simulink model "CartIdentPiMod2"  (R2025b)
settings: Solver=ode1  StartTime=0.0  StopTime=20  FixedStep=0.001  RelTol=1e-3  EnableMultiTasking=on
undefined symbols (not defined in the file): MQTTsample
libraries: raspberrypiCommlib x2, raspberrypiBasiclib x1, simulink x1, raspberrypiIOTlib x1
settings Model: SimulationMode=external  ExtModeTrigMode=oneshot  ExtModeTrigDuration=100000  Creator=Demo11  LastModifiedBy=brfon_9d4n8nc
settings SolverCC: AlgebraicLoopSolver=TrustRegion  PositivePriorityOrder=on  AutoInsertRateTranBlk=on
settings DataIOCC: SaveFormat=Array  SignalLoggingSaveFormat=ModelDataLogs  ReturnWorkspaceOutputs=off  SignalLoggingName=sigsOut
settings OptimizationCC: BlockReduction=off  BooleanDataType=off  EnhancedBackFolding=on  PassReuseOutputArgsAs=Individual arguments  ExpressionDepthLimit=2147483647.0  ZeroExternalMemoryAtStartup=off  ZeroInternalMemoryAtStartup=off  InitFltsAndDblsToZero=on  MaxStackSize=200000  OptimizeBlockOrder=speed  DifferentSizesBufferReuse=on  OptimizationCustomize=off  EfficientTunableParamExpr=on
settings DebuggingCC: SaveWithParameterizedLinksMsg=none  UnderspecifiedInitializationDetection=Classic  MergeDetectMultiDrivingBlocksExec=none  SignalResolutionControl=TryResolveAllWithWarning  MultiTaskDSMMsg=warning  MultiTaskCondExecSysMsg=none  ParameterTunabilityLossMsg=error  FcnCallInpInsideContextMsg=warning  UnconnectedInputMsg=warning  UnconnectedOutputMsg=warning  UnconnectedLineMsg=warning  AllowSymbolicDim=off  StateNameClashWarn=warning  SFUnexpectedBacktrackingDiag=warning  SFNoUnconditionalDefaultTransitionDiag=warning  SFExecutionAtInitializationDiag=none  ArithmeticOperatorsInVariantConditions=warning
settings HardwareCC: ProdBitPerLong=64.0  ProdLargestAtomicInteger=LongLong  ProdLargestAtomicFloat=Double  ProdLongLongMode=on  ProdHWDeviceType=ARM Compatible->ARM Cortex-A (64-bit)  TargetBitPerLong=64.0  TargetBitPerPointer=64.0  TargetIntDivRoundTo=Zero  TargetEndianess=LittleEndian  TargetWordSize=64.0  TargetHWDeviceType=Intel->x86-64
settings ModelReferenceCC: EnableRefExpFcnMdlSchedulingChecks=on  PropagateSignalLabelsOutOfModel=off
settings SFSimCC: SimUseLocalCustomCode=off  CustomCodeUndefinedFunction=UseInterfaceOnly
settings RTWCC: SystemTargetFile=ert.tlc  HardwareBoard=Raspberry Pi (64bit)  TLCOptions="-aInlineSetEventsForThisBaseRateFcn=TLC_FALSE -aSuppressMultiTaskScheduler=TLC_FALSE  -aRateBasedStepFcn=0"  TemplateMakefile=ert_default_tmf  RTWUseLocalCustomCode=off  Toolchain=GNU GCC Embedded Linux  BuildConfiguration=Faster Runs  GPUComputeCapability=3.5  Description=Embedded Coder
settings CodeAppCC: ForceParamTrailComments=on  IgnoreCustomStorageClasses=off  MaxIdLength=95.0  OperatorAnnotations=on  SimulinkDataObjDesc=on  SFDataObjDesc=on  InsertBlockDesc=on
settings ERTTargetCC: ExtModeTransport=2.0  ExtModeStaticAlloc=on  ExtModeMexFile=ext_xcp  ExtModeIntrfLevel=Level2 - Open  InlinedParameterPlacement=Hierarchical  CodeReplacementLibrary=ARM Cortex-A CMSIS  SupportContinuousTime=on  SupportVariableSizeSignals=on
settings ConfigComp: CovMetricSettings=dw  CovSaveCumulativeToWorkspaceVar=on  CovSaveSingleToWorkspaceVar=on  CovExternalEMLEnable=off

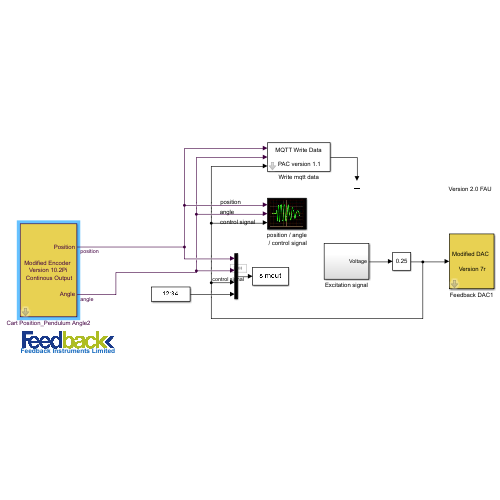
[thumbnail: Simulink's stored preview of the top-level diagram]
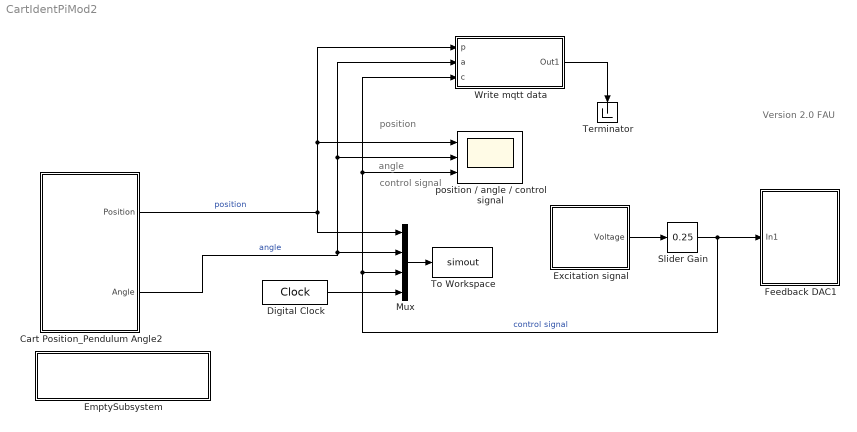
== system CartIdentPiMod2 ==
  note: position
  note: angle
  note: control signal
  note: Version 2.0 FAU
  Cart Position_Pendulum Angle2 : Subsystem  mask(Feedback Encoder Block){st=0.001, of1=0, of2=-1024}
      mask prompts: st "Sample Time"; of1 "Channel 1 Offset"; of2 "Channel 2 Offset"
      mask help: Special block to use with the Feedback experiments to read encoder channels using the digital I/O lines
      mask Display:
      | %image(imread('bckg.bmp'))
      | disp('Modified Encoder \nVersion 10.2Pi\n Continous Output')
      | port_label('output', 1, 'Position')
      | port_label('output', 2, 'Angle')
  Digital Clock : DigitalClock  SampleTime=0.001
  EmptySubsystem : Subsystem
      mask Display:
      | image(imread('FB-inst-blue2.jpg'))
      | disp('\n\nFeedback Instruments Limited')
  Excitation signal : Subsystem
  Feedback DAC1 : Subsystem  mask(DAC Unit for Feedback Experiments){st=0.001, ch=1}
      mask prompts: st "Sample Time"; ch "Output Channel"
      mask help:
      | Digital to Analog Output  for Feedback Experiments
      | using Advantech PCI1711  I/O board
      mask Display:
      | %image(imread('bckg.bmp'))
      | disp('Modified DAC \n\n Version 7r')
  Mux : Mux
  Slider Gain : simulink/Math Operations/Slider Gain  gain=0.25  low=-0.3  high=0.3
  Terminator : Terminator
  To Workspace : ToWorkspace  VariableName=simout  SampleTime=0.05
  Write mqtt data : Subsystem
      mask Display: disp('MQTT Write Data\n\n PAC version 1.1')
  position / angle / control signal : Scope  NumInputPorts=3
      settings: SampleTime=0.001  TimeSpan=20  ActiveDisplayYMinimum=-0.55  ActiveDisplayYMaximum=0.35  DataLoggingMaxPoints=100000  DataLoggingVariableName=ScopeData2
      mask Display: image(imread('scope.jpg'))
  wires:
  Cart Position_Pendulum Angle2/1(Position) -> Write mqtt data/1(p), position / angle / control signal/1, Mux/1  "position"
  Excitation signal/1(Voltage) -> Slider Gain/1
  Cart Position_Pendulum Angle2/2(Angle) -> Write mqtt data/2(a), position / angle / control signal/2, Mux/2  "angle"
  Slider Gain/1 -> Feedback DAC1/1(In1), Mux/3, Write mqtt data/3(c), position / angle / control signal/3  "control signal"
  Mux/1 -> To Workspace/1
  Digital Clock/1 -> Mux/4
  Write mqtt data/1(Out1) -> Terminator/1

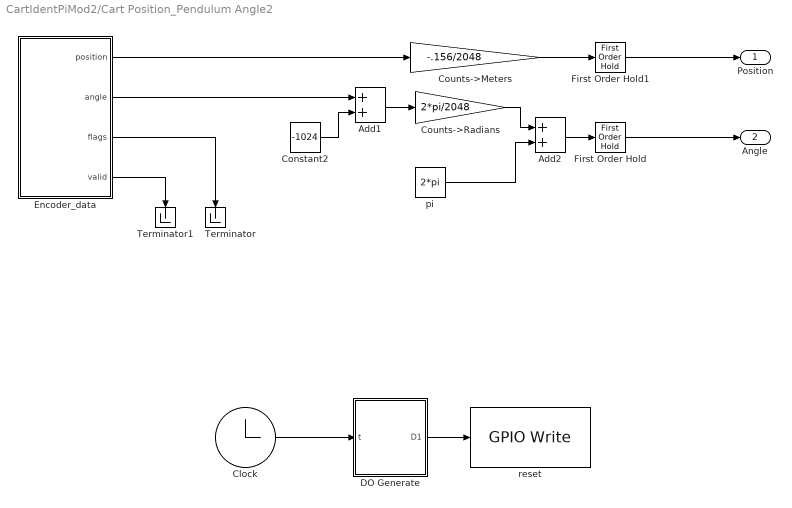
== system CartIdentPiMod2/Cart Position_Pendulum Angle2 ==
  Add1 : Sum
  Add2 : Sum
  Clock : Clock
  Constant2 : Constant  Value=-1024
  Counts->Meters : Gain  Gain=-.156/2048  SaturateOnIntegerOverflow=on  OutDataTypeStr=Inherit: Same as input  ParamDataTypeStr=Inherit: Same as input
  Counts->Radians : Gain  Gain=2*pi/2048  SaturateOnIntegerOverflow=on  OutDataTypeStr=Inherit: Same as input  ParamDataTypeStr=Inherit: Same as input
  DO Generate : MATLAB Function  TreatAsAtomicUnit=on
  Encoder_data : Subsystem
  First Order Hold : FirstOrderHold  OutputAlgorithm=Fast (Minimize Error)  ErrorTolerance=inf
  First Order Hold1 : FirstOrderHold  OutputAlgorithm=Fast (Minimize Error)  ErrorTolerance=inf
  Terminator : Terminator
  Terminator1 : Terminator
  pi : Constant  Value=2*pi
  reset : raspberrypiBasiclib/GPIO Write  BoardProperty=Pi 5 Model  gpio=6  blockPlatform=Raspberry Pi  PinNumber=17  board=[]  direction=[]
  Position : Outport
  Angle : Outport  Port=2
  wires:
  pi/1 -> Add2/2
  Counts->Radians/1 -> Add2/1
  Counts->Meters/1 -> First Order Hold1/1
  Clock/1 -> DO Generate/1(t)
  DO Generate/1(D1) -> reset/1
  Encoder_data/2(angle) -> Add1/1
  Encoder_data/1(position) -> Counts->Meters/1
  Add1/1 -> Counts->Radians/1
  Constant2/1 -> Add1/2
  Encoder_data/4(valid) -> Terminator1/1
  Encoder_data/3(flags) -> Terminator/1
  Add2/1 -> First Order Hold/1
  First Order Hold/1 -> Angle/1
  First Order Hold1/1 -> Position/1

== system CartIdentPiMod2/EmptySubsystem ==

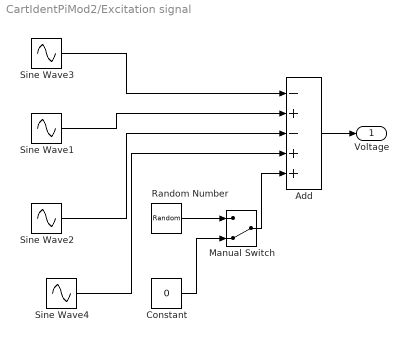
== system CartIdentPiMod2/Excitation signal ==
  Add : Sum  Inputs=-+-++
  Constant : Constant  Value=0
  Manual Switch : ManualSwitch  CurrentSetting=0
  Random Number : RandomNumber  Variance=0.1  SampleTime=0.1
  Sine Wave1 : Sin  Frequency=5  Phase=1  SampleTime=0
  Sine Wave2 : Sin  Frequency=15  SampleTime=0
  Sine Wave3 : Sin  Amplitude=0.5  Phase=0.5  SampleTime=0
  Sine Wave4 : Sin  Frequency=20  Phase=0.3  SampleTime=0
  Voltage : Outport
  wires:
  Add/1 -> Voltage/1
  Sine Wave3/1 -> Add/1
  Sine Wave1/1 -> Add/2
  Sine Wave2/1 -> Add/3
  Sine Wave4/1 -> Add/4
  Random Number/1 -> Manual Switch/1
  Manual Switch/1 -> Add/5
  Constant/1 -> Manual Switch/2

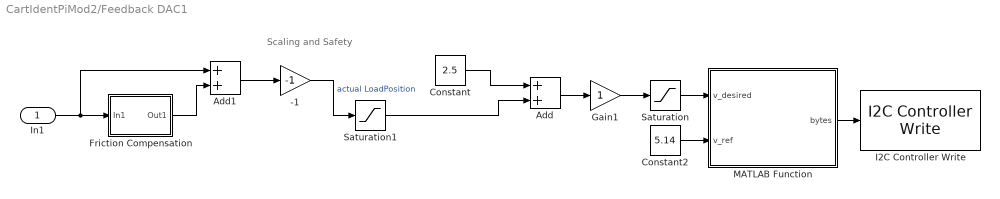
== system CartIdentPiMod2/Feedback DAC1 ==
  note: Scaling and Safety
  In1 : Inport
  -1 : Gain  Gain=-1  SaturateOnIntegerOverflow=on  OutDataTypeStr=Inherit: Same as input  ParamDataTypeStr=Inherit: Same as input
  Add : Sum  OutDataTypeStr=Inherit: Same as first input
  Add1 : Sum
  Constant : Constant  Value=2.5
  Constant2 : Constant  Value=5.14  SampleTime=-1
  Friction Compensation : Subsystem  mask(linear){frictionCompNeg=.1, frictionCompPos=.1}
      mask prompts: frictionCompNeg "Friction Compensation Magnitude in Negative Direction"; frictionCompPos "Friction Compensation Magnitude in Positive Direction"
      mask Display: plot(0,0,100,100,[40,30,20],[87,85,80],[46,54,54,46,46],[90,90,80,80,90],[46,45,45,46,54,55,55,54,46],[78,80,90,91,91,90,80,78,78],[51,51,49,49],[78,10,10,78],[90,80,70,60],[70,80,85,88],[20,10],[80,70],[20,20,15],[73,80,80],[85,80,80],[80,80,74])
  Gain1 : Gain
  I2C Controller Write : raspberrypiCommlib/I2C Controller Write  BoardProperty=Pi 5 Model  I2CModule=1  Mode=Master  SlaveAddress=0x60  SlaveByteOrder=BigEndian  Direction=Transmitter  RegisterAddressMode=off  RegisterAddress=0  SlaveDataType=uint8  DataLength=1  NoAck=off  RepeatedStart=off  OutputStatus=off
  MATLAB Function : MATLAB Function  TreatAsAtomicUnit=on
  Saturation : Saturate  UpperLimit=5.0  LowerLimit=0
  Saturation1 : Saturate  UpperLimit=2.5  LowerLimit=-2.5
  wires:
  MATLAB Function/1(bytes) -> I2C Controller Write/1
  Saturation/1 -> MATLAB Function/1(v_desired)
  Constant2/1 -> MATLAB Function/2(v_ref)
  Add1/1 -> -1/1
  -1/1 -> Saturation1/1  "actual LoadPosition"
  In1/1 -> Add1/1, Friction Compensation/1(In1)
  Friction Compensation/1(Out1) -> Add1/2
  Constant/1 -> Add/1
  Add/1 -> Gain1/1
  Gain1/1 -> Saturation/1
  Saturation1/1 -> Add/2

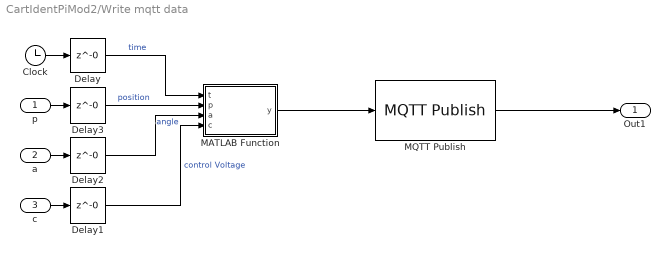
== system CartIdentPiMod2/Write mqtt data ==
  p : Inport
  a : Inport  Port=2
  c : Inport  Port=3
  Clock : Clock
  Delay{,1..3} (4 alike) : Delay  DelayLength=0  InitialCondition=0  SampleTime=MQTTsample
  MATLAB Function : MATLAB Function  TreatAsAtomicUnit=on
  MQTT Publish : raspberrypiIOTlib/MQTT Publish  Topic=raspi/to_django  QoS=0  RetainMsg=off  blockPlatform=RASPBERRYPI
  Out1 : Outport
  wires:
  MQTT Publish/1 -> Out1/1
  a/1 -> Delay2/1
  Clock/1 -> Delay/1
  Delay/1 -> MATLAB Function/1(t)  "time"
  p/1 -> Delay3/1
  Delay2/1 -> MATLAB Function/3(a)  "angle"
  c/1 -> Delay1/1
  Delay1/1 -> MATLAB Function/4(c)  "control Voltage"
  MATLAB Function/1(y) -> MQTT Publish/1
  Delay3/1 -> MATLAB Function/2(p)  "position"

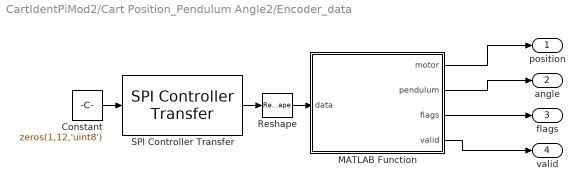
== system CartIdentPiMod2/Cart Position_Pendulum Angle2/Encoder_data ==
  Constant : Constant  Value=zeros(1,12,'uint8')
  MATLAB Function : MATLAB Function  TreatAsAtomicUnit=on
  Reshape : Reshape
  SPI Controller Transfer : raspberrypiCommlib/SPI Controller Transfer  BoardProperty=Pi 5 Model  SSPin=SPI0_CE0  SPIModule=uint32(0)  Mode=Master  BusSpeed=1000000  Pin=uint32(0)  FirstBitToTransfer=Most significant bit (MSB)  ClockMode=1  BlockFunction=Transfer  RegisterAddress=0  OutputDataType=int8  OutputDataLength=1
  position : Outport
  angle : Outport  Port=2
  flags : Outport  Port=3
  valid : Outport  Port=4
  wires:
  Constant/1 -> SPI Controller Transfer/1
  MATLAB Function/3(flags) -> flags/1
  SPI Controller Transfer/1 -> Reshape/1
  Reshape/1 -> MATLAB Function/1(data)
  MATLAB Function/2(pendulum) -> angle/1
  MATLAB Function/4(valid) -> valid/1
  MATLAB Function/1(motor) -> position/1

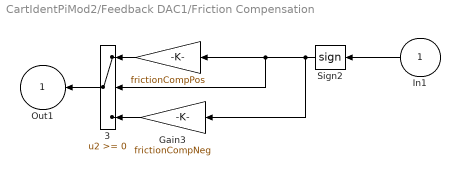
== system CartIdentPiMod2/Feedback DAC1/Friction Compensation ==
  In1 : Inport
  " " : Gain  Gain=frictionCompPos  SaturateOnIntegerOverflow=on  OutDataTypeStr=Inherit: Same as input  ParamDataTypeStr=Inherit: Same as input
  3 : Switch
  Gain3 : Gain  Gain=frictionCompNeg  SaturateOnIntegerOverflow=on  OutDataTypeStr=Inherit: Same as input  ParamDataTypeStr=Inherit: Same as input
  Sign2 : Signum  Tag=T
  Out1 : Outport  InitialOutput=0
  wires:
  3/1 -> Out1/1
  Sign2/1 -> 3/2, " "/1, Gain3/1
  Gain3/1 -> 3/3
  " "/1 -> 3/1
  In1/1 -> Sign2/1

== matlab function CartIdentPiMod2/Cart Position_Pendulum Angle2/DO Generate ==
  data: D1 output; t input
%%pendulum 10
function D1  = generate_DO(t)
    if t <= 0.002
        D1 = 1;  % RESET on first sample
    else
        D1 = 0;
    end
end



%%pendulum 5
% function [D1, D2] = generate_DO(counter, t)
%     if t <= 0.002
%         D1 = 1;  % RESET on first sample
%         % D2 = 0;
%     else
%         D1 = 0;
%     %     D2 = 0;
%         % if mod(counter, 4) < 2
%         %     D1 = 0;
%         %     D2 = 0;
%         % else
%         %     D1 = 1;
%         %     D2 = 0;
%         % end
%     end
% end


%%pendulum 4
% function DO = generate_DO(counter)
%     switch counter
%         case 0
%             DO = 4;  % Reset/idle
%         case 1
%             DO = 1;  % Set DO=1 (ESP32 prepares high byte)
%         case 2
%             DO = 4;  % Keep DO=1 (Simulink reads high byte)        
%         case 3
%             DO = 4;  % Keep DO=1 (Simulink reads high byte)        
%         case 4
%             DO = 2;  % Keep DO=1 (Simulink reads high byte)        
% %         case 3
% %             DO = 1;  % Keep DO=1 (Simulink reads high byte)
% %         case 3
% %             DO = 2; %seperations
% %         case 5
% %             DO = 4; %seperations
% %         case 4
% %             DO = 2;  % Set DO=2 (ESP32 prepares low byte)
% %         case 7
% %             DO = 2;  % Keep DO=2 (Simulink reads low byte)
% %         case 8
% %             DO = 2;  % Keep DO=2 (Simulink reads low byte)
% %         case 9
% %             DO = 4;  % Unlatch
%         otherwise
%             DO = 4;
%     end
% end
% 
% function DO = generate_DO(counter)
%     % Just toggle between 0 and 1
%     if counter == 0
%         DO = 1;  % Motor state
%     else
%         DO = 0;  % Pendulum state
%     end
% end

== matlab function CartIdentPiMod2/Write mqtt data/MATLAB Function ==
  data: t input; p input; y output; a input; c input
function y = fmtstr(t,p,a,c)

y = "{time: "+string(t)+", position: "+string(p)+", angle: "+string(a)+", control: "+string(c)+"}";

== matlab function CartIdentPiMod2/Feedback DAC1/MATLAB Function ==
  data: v_desired input; bytes output; v_ref input
function bytes = voltToMCP4725(v_desired, v_ref)
    % v_desired: desired output voltage (0 to v_ref)
    % v_ref: DAC supply voltage (5.0)
    dacVal = uint16(round((v_desired / v_ref) * 4095));
    dacVal = min(dacVal, uint16(4095));
    b0 = uint8(64);                        % 0x40 command byte
    b1 = uint8(bitshift(dacVal, -4));      % upper 8 bits
    b2 = uint8(bitshift(bitand(dacVal, uint16(15)), 4)); % lower 4 bits
    bytes = [b0; b1; b2];
end

== matlab function CartIdentPiMod2/Cart Position_Pendulum Angle2/Encoder_data/MATLAB Function ==
  data: data input uint8 size=[1 12]; motor output; pendulum output; flags output; valid output
function [motor, pendulum, flags, valid] = unpack_spi(data)

% Checksum
chk = uint8(0);
for i = 1:9
    chk = bitxor(chk, data(i));
end
valid = logical(chk == data(10));

% Motor — bytes 1-4 little-endian
motor_int = int32(data(1)) + ...
        bitshift(int32(data(2)), 8) + ...
        bitshift(int32(data(3)), 16) + ...
        bitshift(int32(data(4)), 24);

% Pendulum — bytes 5-8 little-endian
pend_int = int32(data(5)) + ...
           bitshift(int32(data(6)), 8) + ...
           bitshift(int32(data(7)), 16) + ...
           bitshift(int32(data(8)), 24);

% Flags
flags = uint8(data(9));

% Output as single (32-bit float) for use in control blocks
motor    = double(motor_int);
pendulum = single(pend_int);

end
